simulink model "model_AERO2_simul_R2021a"  (R2021a)
settings: Solver=ode1  StartTime=0.0  StopTime=tmax  FixedStep=Ts  RelTol=1e-3
InitFcn:
  | if ~exist('Kp','var') || ~exist('meas_on','var'), nlc_setup; end
values from neighbouring files (symbols this model uses):
  meas_on = 1    [model_AERO2_simul_ini.m]
  Ts = 0.002    [model_AERO2_simul_ini.m]
settings Model: ExtModeTrigDuration=20000  Creator=MLevis  LastModifiedBy=ramon
settings DataIOCC: SaveOutput=off  SignalLogging=off  SaveTime=off  ReturnWorkspaceOutputs=off
settings DebuggingCC: UnderspecifiedInitializationDetection=Classic  MergeDetectMultiDrivingBlocksExec=none  UnconnectedInputMsg=none  UnconnectedOutputMsg=none  UnconnectedLineMsg=none
settings ModelReferenceCC: EnableRefExpFcnMdlSchedulingChecks=off  PropagateSignalLabelsOutOfModel=off
settings RTWCC: Description=Generic Real-Time Target  GPUComputeCapability=5.0  DLArmComputeVersion=20.02.1
settings ConfigComp: CovBoundaryAbsTol=1.0e-5

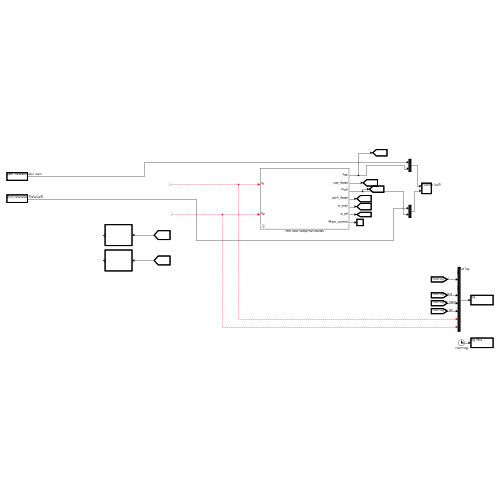
[thumbnail: Simulink's stored preview of the top-level diagram]
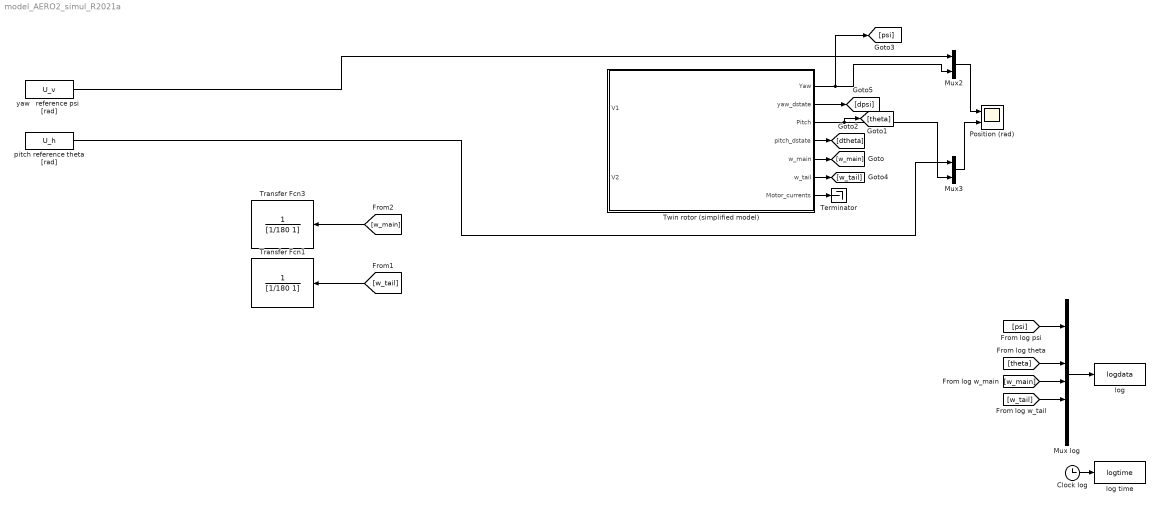
== system model_AERO2_simul_R2021a ==
  Clock log : Clock
  Mux log : Mux  Inputs=8
  Mux2 : Mux  Inputs=2
  Mux3 : Mux  Inputs=2
  Position (rad) : Scope  NumInputPorts=2
  Terminator : Terminator
  Transfer Fcn1 : TransferFcn  Denominator=[1/180 1]
  Transfer Fcn3 : TransferFcn  Denominator=[1/180 1]
  Twin rotor (simplified model) : Subsystem  mask{meas=meas_on}
      mask prompts: meas "Measurement effects (1 = encoder quantization + sensor noise, 0 = ideal)"
      mask help: Simplified twin-rotor model (eq. (simp) of twin_rotor_FL_merged.tex) with DC-motor rotor dynamics. Inputs: V1 main-rotor voltage, V2 tail-rotor voltage [V]. Outputs: same signals as the QUARC interface of lin_feedback_v1.slx, continuous (no zero-order holds; sensor noise generated at Ts).
  log : ToWorkspace  VariableName=logdata  SampleTime=Ts
  log time : ToWorkspace  VariableName=logtime  SampleTime=Ts
  pitch reference theta [rad] : FromWorkspace  VariableName=U_h  OutputAfterFinalValue=Setting to zero
  yaw   reference psi  [rad] : FromWorkspace  VariableName=U_v  OutputAfterFinalValue=Setting to zero
  wires:
  [w_main] -> Transfer Fcn3/1
  [w_tail] -> Transfer Fcn1/1
  Mux2/1 -> Position (rad)/1
  Mux3/1 -> Position (rad)/2
  [psi] -> Mux log/2
  [theta] -> Mux log/4
  [w_main] -> Mux log/5
  [w_tail] -> Mux log/6
  Mux log/1 -> log/1
  Clock log/1 -> log time/1
  Twin rotor (simplified model)/7(Motor_currents) -> Terminator/1
  Twin rotor (simplified model)/3(Pitch) -> [theta], Mux3/2
  Twin rotor (simplified model)/1(Yaw) -> [psi], Mux2/2
  Twin rotor (simplified model)/4(pitch_dstate) -> [dtheta]
  Twin rotor (simplified model)/5(w_main) -> [w_main]
  Twin rotor (simplified model)/6(w_tail) -> [w_tail]
  Twin rotor (simplified model)/2(yaw_dstate) -> [dpsi]
  ? -> Mux log/7, Twin rotor (simplified model)/1(V1)
  ? -> Mux log/8, Twin rotor (simplified model)/2(V2)
  yaw   reference psi  [rad]/1 -> Mux2/1
  pitch reference theta [rad]/1 -> Mux3/1

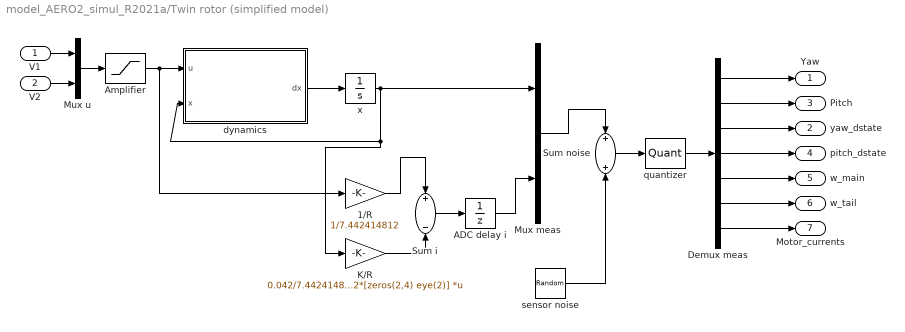
== system model_AERO2_simul_R2021a/Twin rotor (simplified model) ==
  V1 : Inport
  V2 : Inport  Port=2
  1/R : Gain  Gain=1/7.442414812
  ADC delay i : UnitDelay  InitialCondition=[0;0]  SampleTime=0.002
  Amplifier : Saturate  UpperLimit=24  LowerLimit=-24
  Demux meas : Demux  Outputs=[1 1 1 1 1 1 2]
  K/R : Gain  Gain=0.042/7.442414812*[zeros(2,4) eye(2)]  Multiplication=Matrix(K*u)
  Mux meas : Mux  Inputs=[6 2]
  Mux u : Mux  Inputs=2
  Sum i : Sum  Inputs=+-
  Sum noise : Sum
  dynamics : MATLAB Function  TreatAsAtomicUnit=on
  quantizer : Quantizer  QuantizationInterval=max((meas)*[0.0015339807878856412;0.0030679615757712823;0.001;0.001;0.050000000000000003;0.050000000000000003;0.001;0.001], 1e-12)
  sensor noise : RandomNumber  Mean=zeros(8,1)  Variance=((meas)*[0.0005;0.0005;0.005;0.005;0.3;0.3;0.01;0.01]).^2  Seed=[61027;18839;4421;30893;23341;7781;51117;9013]  SampleTime=0.002
  x : Integrator  InitialCondition=zeros(6,1)
  Yaw : Outport
  yaw_dstate : Outport  Port=2
  Pitch : Outport  Port=3
  pitch_dstate : Outport  Port=4
  w_main : Outport  Port=5
  w_tail : Outport  Port=6
  Motor_currents : Outport  Port=7
  wires:
  V1/1 -> Mux u/1
  V2/1 -> Mux u/2
  Mux u/1 -> Amplifier/1
  Amplifier/1 -> dynamics/1(u), 1/R/1
  dynamics/1(dx) -> x/1
  x/1 -> Mux meas/1, dynamics/2(x), K/R/1
  1/R/1 -> Sum i/1
  K/R/1 -> Sum i/2
  Sum i/1 -> ADC delay i/1
  ADC delay i/1 -> Mux meas/2
  Mux meas/1 -> Sum noise/1
  sensor noise/1 -> Sum noise/2
  Sum noise/1 -> quantizer/1
  quantizer/1 -> Demux meas/1
  Demux meas/1 -> Yaw/1
  Demux meas/3 -> yaw_dstate/1
  Demux meas/2 -> Pitch/1
  Demux meas/4 -> pitch_dstate/1
  Demux meas/5 -> w_main/1
  Demux meas/6 -> w_tail/1
  Demux meas/7 -> Motor_currents/1

== matlab function model_AERO2_simul_R2021a/Twin rotor (simplified model)/dynamics ==
  data: u input; dx output; x input
function dx = fcn(u, x)
%% Simplified twin-rotor model of aero2_model.pdf (2-DOF body + first-order motors)
p = struct('Jph', 0.64070000000000005, ...
    'jph', 0.01, ...
    'Jth', 0.71640000000000004, ...
    'G', 0.025399999999999999, ...
    'kT', 4.2486999999999997e-06, ...
    'kF', 2.5525999999999999e-05, ...
    'L', 0.16700000000000001, ...
    'Cor', 0.63070000000000004, ...
    'Dph', 0, ...
    'Dth', 0, ...
    'aw', 5.7800000000000002, ...
    'bw', 96.531999999999996);
dx = tr_simp_dyn(x, u, p);
end

function dx = tr_simp_dyn(x, u, p)
%TR_SIMP_DYN  Simplified twin-rotor model with voltage inputs (aero2_model.pdf).
%   Body: reduced 2-DOF model, eq. (simp)
%     Mq(th) [ddpsi; ddth] + cq + Bq dq + gq = Gamma(th) [wm|wm|; wt|wt|]
%   with cq = [-Cor sin(2th) dth dpsi; 1/2 Cor sin(2th) dpsi^2]
%   (no gyroscopic coupling, no motor reaction channel, s_m=+1, s_t=-1).
%   Rotors: first-order motor model of the hand-out
%     dw = -aw w + bw v
%   State x = [psi, theta, dpsi, dtheta, wm, wt], input u = [Um, Ut].
%   p: Jph jph Jth Dph Dth Cor L G kF kT aw bw (psim of tr_instructor_params).

    th = x(2);  dps = x(3);  dth = x(4);
    c = cos(th);  s = sin(th);
    tau = [x(5)*abs(x(5)); x(6)*abs(x(6))];

    Ms  = [p.Jph*c^2 + p.jph*s^2, 0; 0, p.Jth];
    Cs  = [-p.Cor*sin(2*th)*dth*dps; 0.5*p.Cor*sin(2*th)*dps^2];
    Ds  = [p.Dph*dps; p.Dth*dth];
    Gs  = [0; p.G*s];
    Gam = [c 0; 0 1]*[-p.kT, p.L*p.kF; p.L*p.kF, p.kT];
    ddq = Ms\(Gam*tau - Cs - Ds - Gs);

    dw  = -p.aw*x(5:6) + p.bw*u(:);
    dx  = [x(3:4); ddq; dw];
end
